simulink model "sens_lidar_model"  (R2026b)
settings: Solver=VariableStepAuto
values from neighbouring files (symbols this model uses):
  P = (P + P.')/2    [sens_nav_ekf.m]
undefined symbols (not defined in the file or in its folder): sens_lidar2d_fast_prm, Ts
libraries: uavsimlib x3
settings Model: Creator=aomar  LastModifiedBy=aomar

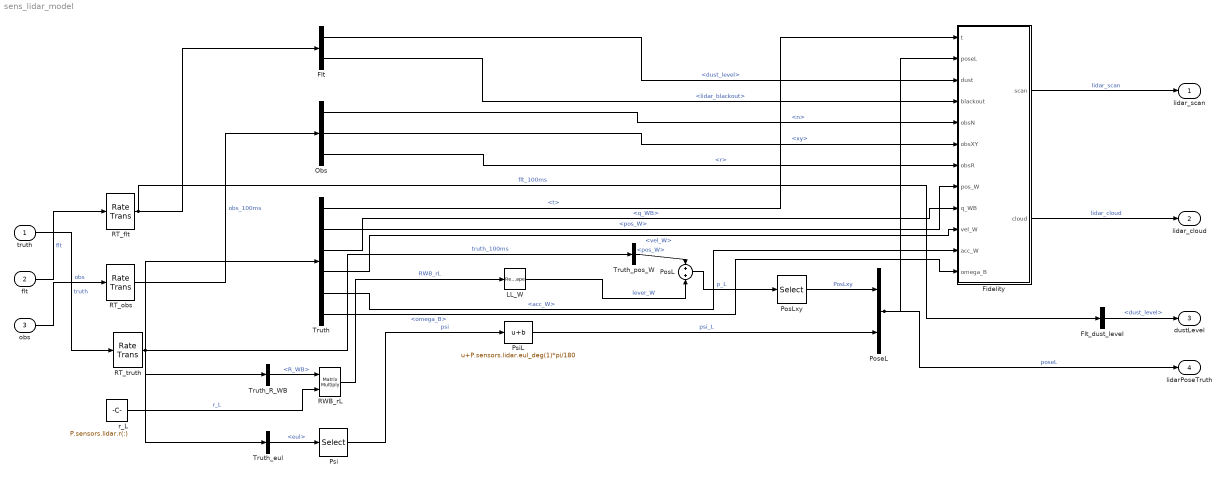
== system sens_lidar_model ==
  truth : Inport  OutDataTypeStr=Bus: Bus_TruthState  SampleTime=Ts.base
  flt : Inport  Port=2  OutDataTypeStr=Bus: Bus_FaultInject  SampleTime=Ts.ctrl
  obs : Inport  Port=3  OutDataTypeStr=Bus: Bus_ObstaclesDyn  SampleTime=Ts.ctrl
  Fidelity : Subsystem  Variant=on
  Flt : BusSelector  OutputSignals=dust_level,lidar_blackout
  Flt_dust_level : BusSelector  OutputSignals=dust_level
  LL_W : Reshape
  Obs : BusSelector  OutputSignals=n,xy,r
  PosL : Sum
  PosLxy : Selector  InputPortWidth=3  IndexOptions=Index vector (dialog)  Indices=[1 2]  OutputSizes=1
  PoseL : Mux  Inputs=[2 1]
  Psi : Selector  InputPortWidth=3  IndexOptions=Index vector (dialog)  Indices=1  OutputSizes=1
  PsiL : Bias  Bias=P.sensors.lidar.eul_deg(1)*pi/180  SaturateOnIntegerOverflow=off
  RT_flt : RateTransition  OutPortSampleTime=Ts.lidar
  RT_obs : RateTransition  OutPortSampleTime=Ts.lidar
  RT_truth : RateTransition  OutPortSampleTime=Ts.lidar
  RWB_rL : Product  Multiplication=Matrix(*)
  Truth : BusSelector  OutputSignals=t,pos_W,q_WB,vel_W,acc_W,omega_B
  Truth_R_WB : BusSelector  OutputSignals=R_WB
  Truth_eul : BusSelector  OutputSignals=eul
  Truth_pos_W : BusSelector  OutputSignals=pos_W
  r_L : Constant  Value=P.sensors.lidar.r(:)  VectorParams1D=off
  lidar_scan : Outport  OutDataTypeStr=Bus: Bus_LidarScanRaw
  lidar_cloud : Outport  Port=2  OutDataTypeStr=Bus: Bus_LidarCloudRaw
  dustLevel : Outport  Port=3  OutDataTypeStr=double
  lidarPoseTruth : Outport  Port=4  OutDataTypeStr=double
  wires:
  truth/1 -> RT_truth/1  "truth"
  flt/1 -> RT_flt/1  "flt"
  obs/1 -> RT_obs/1  "obs"
  r_L/1 -> RWB_rL/2  "r_L"
  RT_flt/1 -> Flt/1, Flt_dust_level/1  "flt_100ms"
  RT_obs/1 -> Obs/1  "obs_100ms"
  RT_truth/1 -> Truth_pos_W/1, Truth_eul/1, Truth/1, Truth_R_WB/1  "truth_100ms"
  Truth_R_WB/1 -> RWB_rL/1  "<R_WB>"
  Truth_eul/1 -> Psi/1  "<eul>"
  Flt/1 -> Fidelity/3(dust)  "<dust_level>"
  Flt/2 -> Fidelity/4(blackout)  "<lidar_blackout>"
  Obs/1 -> Fidelity/5(obsN)  "<n>"
  Obs/2 -> Fidelity/6(obsXY)  "<xy>"
  Obs/3 -> Fidelity/7(obsR)  "<r>"
  Truth/1 -> Fidelity/1(t)  "<t>"
  Truth/2 -> Fidelity/8(pos_W)  "<pos_W>"
  Truth/3 -> Fidelity/9(q_WB)  "<q_WB>"
  Truth/4 -> Fidelity/10(vel_W)  "<vel_W>"
  Truth/5 -> Fidelity/11(acc_W)  "<acc_W>"
  Truth/6 -> Fidelity/12(omega_B)  "<omega_B>"
  RWB_rL/1 -> LL_W/1  "RWB_rL"
  Psi/1 -> PsiL/1  "psi"
  LL_W/1 -> PosL/2  "lever_W"
  PsiL/1 -> PoseL/2  "psi_L"
  Truth_pos_W/1 -> PosL/1  "<pos_W>"
  PosL/1 -> PosLxy/1  "p_L"
  PosLxy/1 -> PoseL/1  "PosLxy"
  PoseL/1 -> Fidelity/2(poseL), lidarPoseTruth/1  "poseL"
  Fidelity/1(scan) -> lidar_scan/1  "lidar_scan"
  Fidelity/2(cloud) -> lidar_cloud/1  "lidar_cloud"
  Flt_dust_level/1 -> dustLevel/1  "<dust_level>"

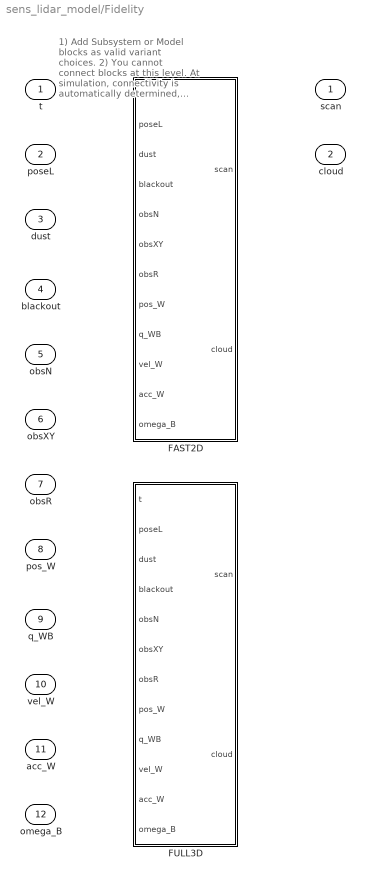
== system sens_lidar_model/Fidelity ==
  note: 1) Add Subsystem or Model blocks as valid variant choices.
      | 2) You cannot connect blocks at this level. At simulation, connectivity is automatically
      | determined, based on the active variant and port name matching.
  t : Inport
  poseL : Inport  Port=2
  dust : Inport  Port=3
  blackout : Inport  Port=4
  obsN : Inport  Port=5
  obsXY : Inport  Port=6
  obsR : Inport  Port=7
  pos_W : Inport  Port=8
  q_WB : Inport  Port=9
  vel_W : Inport  Port=10
  acc_W : Inport  Port=11
  omega_B : Inport  Port=12
  FAST2D : Subsystem  Description=FAST2D (VC_LIDAR == 1): 360-beam height-band scan, lidar_cloud = P.ic.Bus_LidarCloudRaw.  VariantControl=VC_LIDAR == 1
  FULL3D : Subsystem  Description=FULL3D (VC_LIDAR == 2): uavScenario sens_uavScene (base), platform Shaddad with sensor Lidar; organised cloud padded with NaN to [32 1024 3]; lidar_scan = P.ic.Bus_LidarScanRaw. Interpreted only.  VariantControl=VC_LIDAR == 2
  scan : Outport
  cloud : Outport  Port=2

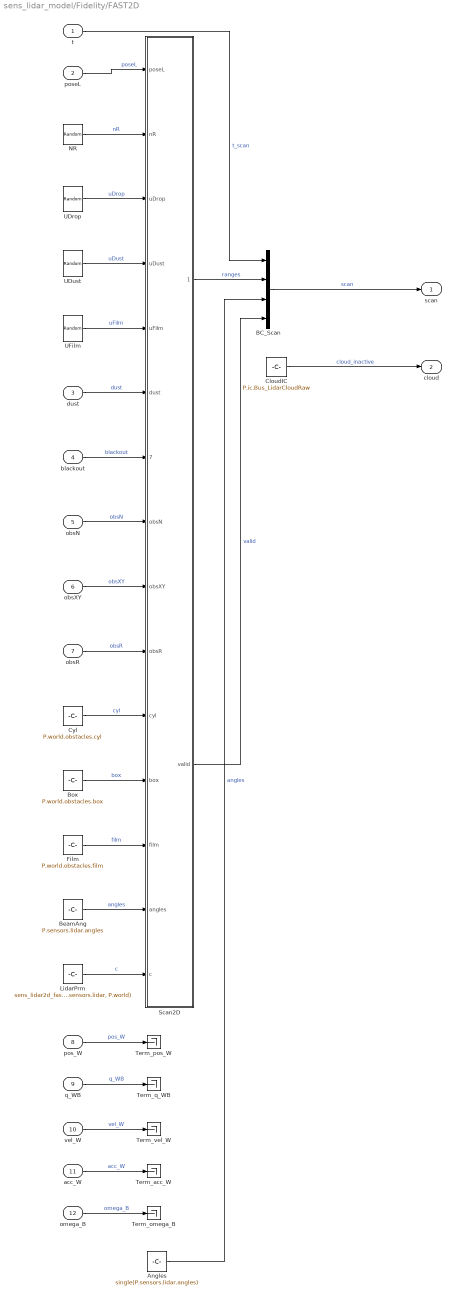
== system sens_lidar_model/Fidelity/FAST2D ==
  t : Inport
  poseL : Inport  Port=2
  dust : Inport  Port=3
  blackout : Inport  Port=4
  obsN : Inport  Port=5
  obsXY : Inport  Port=6
  obsR : Inport  Port=7
  pos_W : Inport  Port=8
  q_WB : Inport  Port=9
  vel_W : Inport  Port=10
  acc_W : Inport  Port=11
  omega_B : Inport  Port=12
  Angles : Constant  Value=single(P.sensors.lidar.angles)  OutDataTypeStr=single  SampleTime=Ts.lidar
  BC_Scan : BusCreator  Inputs=4  OutDataTypeStr=Bus: Bus_LidarScanRaw  NonVirtualBus=on
      settings: InheritFromInputs=off
  BeamAng : Constant  Value=P.sensors.lidar.angles  VectorParams1D=off
  Box : Constant  Value=P.world.obstacles.box  VectorParams1D=off
  CloudIC : Constant  Value=P.ic.Bus_LidarCloudRaw  OutDataTypeStr=Bus: Bus_LidarCloudRaw  SampleTime=Ts.lidar
  Cyl : Constant  Value=P.world.obstacles.cyl  VectorParams1D=off
  Film : Constant  Value=P.world.obstacles.film  VectorParams1D=off
  LidarPrm : Constant  Value=sens_lidar2d_fast_prm(P.sensors.lidar, P.world)  VectorParams1D=off
  NR : RandomNumber  Mean=zeros(1,P.sensors.lidar.nBeams)  Variance=ones(1,P.sensors.lidar.nBeams)  Seed=P.sensors.lidar.seedNR  SampleTime=Ts.lidar
  Scan2D : MATLAB Function  TreatAsAtomicUnit=on
  Term_acc_W : Terminator
  Term_omega_B : Terminator
  Term_pos_W : Terminator
  Term_q_WB : Terminator
  Term_vel_W : Terminator
  UDrop : UniformRandomNumber  Minimum=zeros(1,P.sensors.lidar.nBeams)  Maximum=ones(1,P.sensors.lidar.nBeams)  Seed=P.sensors.lidar.seedDrop  SampleTime=Ts.lidar
  UDust : UniformRandomNumber  Minimum=zeros(1,P.sensors.lidar.nBeams)  Maximum=ones(1,P.sensors.lidar.nBeams)  Seed=P.sensors.lidar.seedDust  SampleTime=Ts.lidar
  UFilm : UniformRandomNumber  Minimum=zeros(1,P.sensors.lidar.nBeams)  Maximum=ones(1,P.sensors.lidar.nBeams)  Seed=P.sensors.lidar.seedFilm  SampleTime=Ts.lidar
  scan : Outport
  cloud : Outport  Port=2
  wires:
  t/1 -> BC_Scan/1  "t_scan"
  poseL/1 -> Scan2D/1(poseL)  "poseL"
  NR/1 -> Scan2D/2(nR)  "nR"
  UDrop/1 -> Scan2D/3(uDrop)  "uDrop"
  UDust/1 -> Scan2D/4(uDust)  "uDust"
  UFilm/1 -> Scan2D/5(uFilm)  "uFilm"
  dust/1 -> Scan2D/6(dust)  "dust"
  blackout/1 -> Scan2D/7(blackout)  "blackout"
  obsN/1 -> Scan2D/8(obsN)  "obsN"
  obsXY/1 -> Scan2D/9(obsXY)  "obsXY"
  obsR/1 -> Scan2D/10(obsR)  "obsR"
  Cyl/1 -> Scan2D/11(cyl)  "cyl"
  Box/1 -> Scan2D/12(box)  "box"
  Film/1 -> Scan2D/13(film)  "film"
  BeamAng/1 -> Scan2D/14(angles)  "angles"
  LidarPrm/1 -> Scan2D/15(c)  "c"
  pos_W/1 -> Term_pos_W/1  "pos_W"
  q_WB/1 -> Term_q_WB/1  "q_WB"
  vel_W/1 -> Term_vel_W/1  "vel_W"
  acc_W/1 -> Term_acc_W/1  "acc_W"
  omega_B/1 -> Term_omega_B/1  "omega_B"
  Angles/1 -> BC_Scan/3  "angles"
  Scan2D/1(ranges) -> BC_Scan/2  "ranges"
  Scan2D/2(valid) -> BC_Scan/4  "valid"
  BC_Scan/1 -> scan/1  "scan"
  CloudIC/1 -> cloud/1  "cloud_inactive"

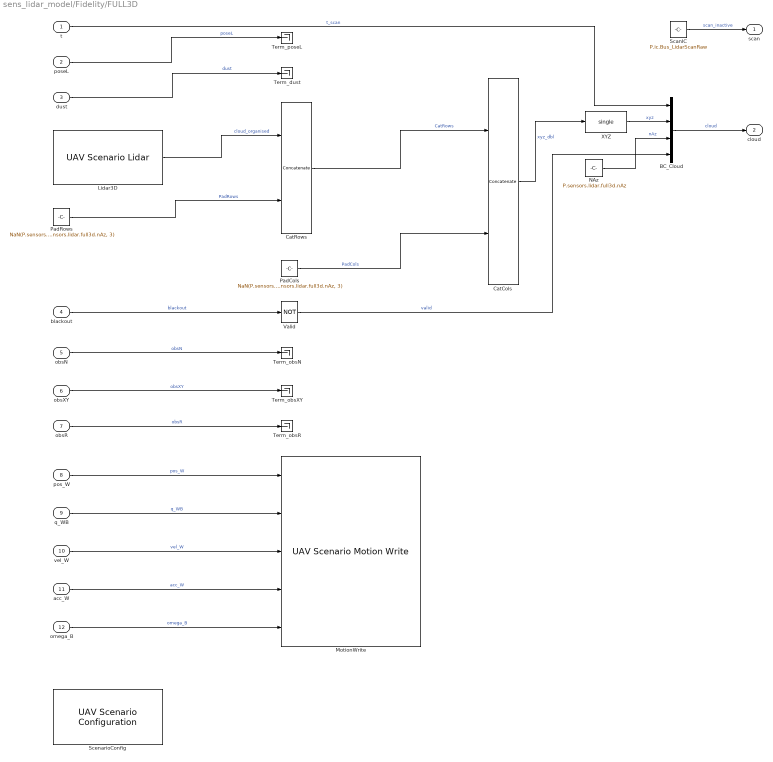
== system sens_lidar_model/Fidelity/FULL3D ==
  t : Inport
  poseL : Inport  Port=2
  dust : Inport  Port=3
  blackout : Inport  Port=4
  obsN : Inport  Port=5
  obsXY : Inport  Port=6
  obsR : Inport  Port=7
  pos_W : Inport  Port=8
  q_WB : Inport  Port=9
  vel_W : Inport  Port=10
  acc_W : Inport  Port=11
  omega_B : Inport  Port=12
  BC_Cloud : BusCreator  Inputs=4  OutDataTypeStr=Bus: Bus_LidarCloudRaw  NonVirtualBus=on
      settings: InheritFromInputs=off
  CatCols : Concatenate  Mode=Multidimensional array  ConcatenateDimension=2
  CatRows : Concatenate  Mode=Multidimensional array
  Lidar3D : uavsimlib/UAV Scenario Lidar  Priority=1  SensorName=Shaddad/Lidar  MaxRange=P.sensors.lidar.full3d.MaxRange  RangeAccuracy=P.sensors.lidar.full3d.RangeAccuracy  AzimuthLimits=P.sensors.lidar.full3d.AzimuthLimits  AzimuthResolution=P.sensors.lidar.full3d.AzimuthResolution  ElevationLimits=P.sensors.lidar.full3d.ElevationLimits  ElevationResolution=P.sensors.lidar.full3d.ElevationResolution  HasNoise=on  HasOrganizedOutput=on  SampleTime=Ts.lidar
  MotionWrite : uavsimlib/UAV Scenario Motion Write  Priority=0  PlatName='Shaddad'  ReferenceFrame=ENU
  NAz : Constant  Value=P.sensors.lidar.full3d.nAz  OutDataTypeStr=uint16  SampleTime=Ts.lidar
  PadCols : Constant  Value=NaN(P.sensors.lidar.cloudSize(1), P.sensors.lidar.cloudSize(2) - P.sensors.lidar.full3d.nAz, 3)  SampleTime=Ts.lidar
  PadRows : Constant  Value=NaN(P.sensors.lidar.cloudSize(1) - P.sensors.lidar.full3d.nEl, P.sensors.lidar.full3d.nAz, 3)  SampleTime=Ts.lidar
  ScanIC : Constant  Value=P.ic.Bus_LidarScanRaw  OutDataTypeStr=Bus: Bus_LidarScanRaw  SampleTime=Ts.lidar
  ScenarioConfig : uavsimlib/UAV Scenario Configuration  Priority=-1  UAVScenarioObject=sens_uavScene  SampleTime=Ts.lidar  UpdateParam=false  SensorMotionBusName='SensorMotionBus'  PlatformMotionBusName='PlatformMotionBus'  ScenarioMotionBusName='ScenarioMotionBus'  ScenarioMotionSignalName='ScenarioMotions'
  Term_dust : Terminator
  Term_obsN : Terminator
  Term_obsR : Terminator
  Term_obsXY : Terminator
  Term_poseL : Terminator
  Valid : Logic  Operator=NOT  Inputs=1  AllPortsSameDT=off  OutDataTypeStr=boolean
  XYZ : DataTypeConversion  OutDataTypeStr=single  RndMeth=Nearest  SaturateOnIntegerOverflow=off
  scan : Outport
  cloud : Outport  Port=2
  wires:
  t/1 -> BC_Cloud/1  "t_scan"
  poseL/1 -> Term_poseL/1  "poseL"
  dust/1 -> Term_dust/1  "dust"
  PadRows/1 -> CatRows/2  "PadRows"
  blackout/1 -> Valid/1  "blackout"
  obsN/1 -> Term_obsN/1  "obsN"
  obsXY/1 -> Term_obsXY/1  "obsXY"
  obsR/1 -> Term_obsR/1  "obsR"
  pos_W/1 -> MotionWrite/1  "pos_W"
  q_WB/1 -> MotionWrite/2  "q_WB"
  vel_W/1 -> MotionWrite/3  "vel_W"
  acc_W/1 -> MotionWrite/4  "acc_W"
  omega_B/1 -> MotionWrite/5  "omega_B"
  Lidar3D/1 -> CatRows/1  "cloud_organised"
  PadCols/1 -> CatCols/2  "PadCols"
  Valid/1 -> BC_Cloud/4  "valid"
  CatRows/1 -> CatCols/1  "CatRows"
  CatCols/1 -> XYZ/1  "xyz_dbl"
  NAz/1 -> BC_Cloud/3  "nAz"
  XYZ/1 -> BC_Cloud/2  "xyz"
  BC_Cloud/1 -> cloud/1  "cloud"
  ScanIC/1 -> scan/1  "scan_inactive"

== matlab function sens_lidar_model/Fidelity/FAST2D/Scan2D ==
  settings: description=FAST2D height-band ray casting (sensors spec 3.4, F3): subsystems/sensors/sens_lidar2d_fast.m; constants on inputs 11..15 (P.world.obstacles.cyl/box/film, P.sensors.lidar.angles, sens_lidar2d_fast_prm(P.sensors.lidar, P.world))
  data: poseL input; ranges output; nR input; uDrop input; uDust input; uFilm input; dust input; blackout input; obsN input; obsXY input; obsR input; cyl input; box input; film input; angles input; c input; valid output
function [ranges, valid] = fcn(poseL, nR, uDrop, uDust, uFilm, dust, blackout, obsN, obsXY, obsR, cyl, box, film, angles, c)
%#codegen
[ranges, valid] = sens_lidar2d_fast(poseL, nR, uDrop, uDust, uFilm, dust, blackout, obsN, obsXY, obsR, cyl, box, film, angles, c);
